simulink model "sensores_reales_LU"  (R2026b)
settings: Solver=VariableStepAuto
settings Model: Creator=lamun  LastModifiedBy=lamun

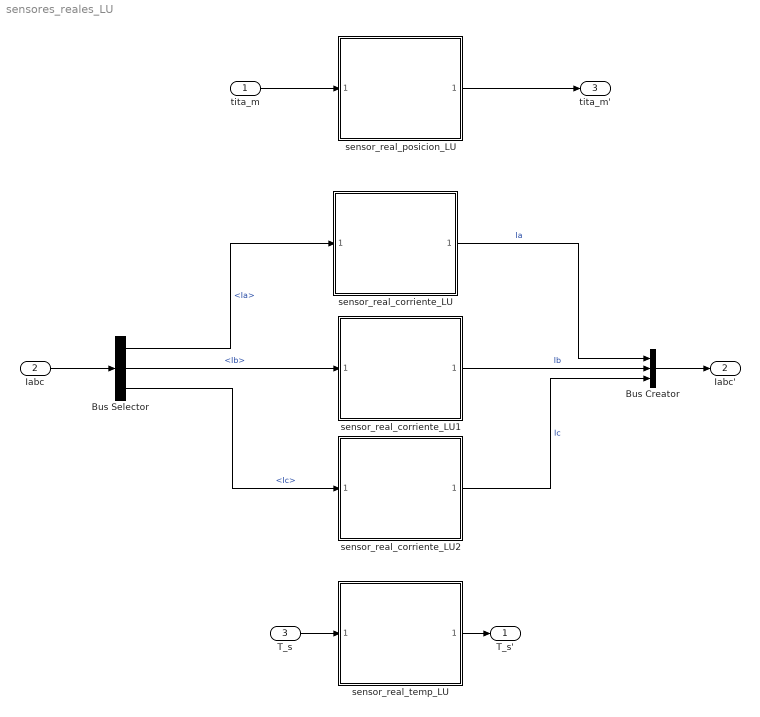
== system sensores_reales_LU ==
  tita_m : Inport
  Iabc : Inport  Port=2
  T_s : Inport  Port=3
  Bus Creator : BusCreator  Inputs=3
  Bus Selector : BusSelector  OutputSignals=Ia,Ib,Ic
  sensor_real_corriente_LU : Subsystem  ReferencedSubsystem=sensor_real_corriente_LU
  sensor_real_corriente_LU1 : Subsystem  ReferencedSubsystem=sensor_real_corriente_LU
  sensor_real_corriente_LU2 : Subsystem  ReferencedSubsystem=sensor_real_corriente_LU
  sensor_real_posicion_LU : Subsystem  ReferencedSubsystem=sensor_real_posicion_LU
  sensor_real_temp_LU : Subsystem  ReferencedSubsystem=sensor_real_temp_LU
  T_s' : Outport
  Iabc' : Outport  Port=2
  tita_m' : Outport  Port=3
  wires:
  tita_m/1 -> sensor_real_posicion_LU/1
  Iabc/1 -> Bus Selector/1
  T_s/1 -> sensor_real_temp_LU/1
  sensor_real_temp_LU/1 -> T_s'/1
  sensor_real_corriente_LU/1 -> Bus Creator/1  "Ia"
  sensor_real_corriente_LU1/1 -> Bus Creator/2  "Ib"
  sensor_real_corriente_LU2/1 -> Bus Creator/3  "Ic"
  Bus Creator/1 -> Iabc'/1
  sensor_real_posicion_LU/1 -> tita_m'/1
  Bus Selector/1 -> sensor_real_corriente_LU/1  "<Ia>"
  Bus Selector/2 -> sensor_real_corriente_LU1/1  "<Ib>"
  Bus Selector/3 -> sensor_real_corriente_LU2/1  "<Ic>"
